simulink model "foc_im_spwm"  (R2024b)
settings: Solver=FixedStepDiscrete  StartTime=0.0  StopTime=P.T_end  FixedStep=P.Ts_power  RelTol=1e-3
values from neighbouring files (symbols this model uses):
  P = motor_params()    [compare_foc_pwm.m]
undefined symbols (not defined in the file or in its folder): DiscIntNeverNeededParam
libraries: slpidlib x3, spsCurrentMeasurementLib x2, spsGroundLib x1, spsabctodq0Lib x1, spsdq0toabcLib x1, spsAsynchronousMachineSIUnitsLib x1, spsUniversalBridgeLib x1, spsDCVoltageSourceLib x1, spspowerguiLib x1
settings Model: Creator=khali  LastModifiedBy=Khalil
settings SolverCC: AutoInsertRateTranBlk=on

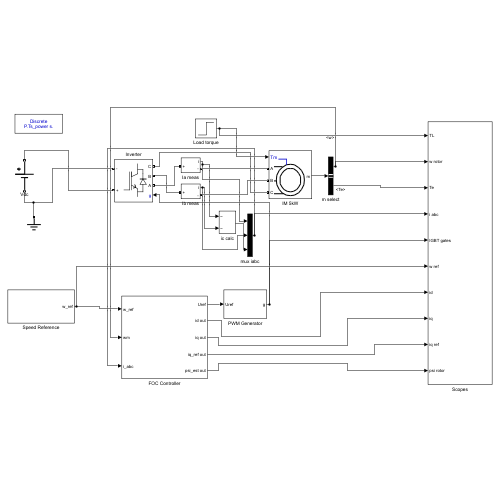
[thumbnail: Simulink's stored preview of the top-level diagram]
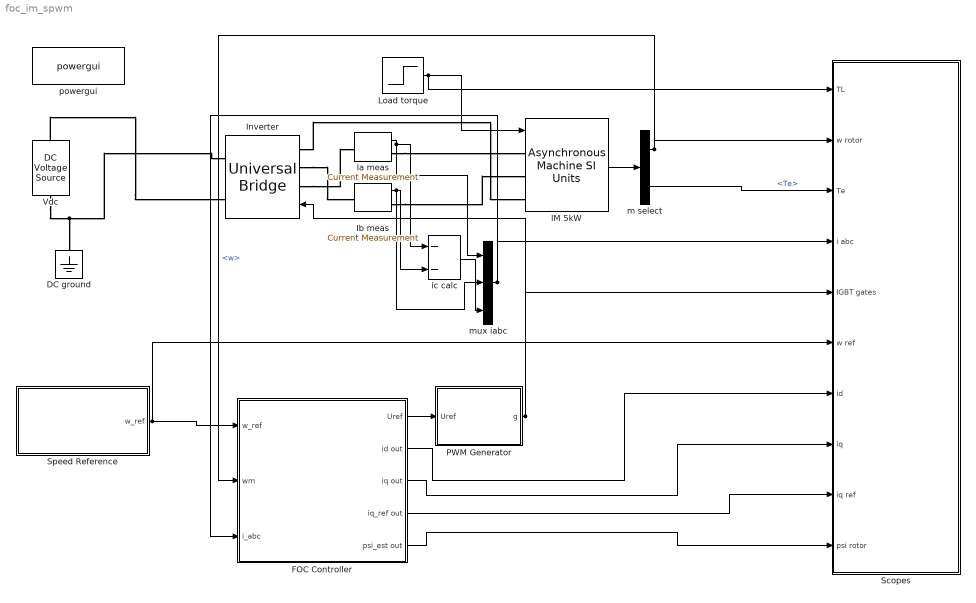
== system foc_im_spwm ==
  DC ground : spsGroundLib/Ground  LConnTagsString=a
  FOC Controller : Subsystem
  IM 5kW : spsAsynchronousMachineSIUnitsLib/Asynchronous Machine SI Units  RotorType=Squirrel-cage  PresetModel=No  MechanicalLoad=Torque Tm  ShowDetailedParameters=on  ReferenceFrame=Rotor  Units=SI  MeasurementBus=on  NominalParameters=[P.Pn P.Vn P.fn]  VoltageRatio=1  Stator=[P.Rs P.Lls]  Rotor=[P.Rr P.Llr]  Cage1=[0.4155 0.002066]  Cage2=[0.4168 0.0003495]  Lm=P.Lm  Mechanical=[P.J P.B P.p]  PolePairs=2  InitialConditions=[1 0 0 0 0 0 0 0]  SimulateSaturation=off  Saturation=[14.03593122, 27.81365428, 53.79336849, 72.68890987, 97.98006896, 148.6815601, 215.7428561, 302.9841135, 428.7778367 ; 230, 322, 414, 460, 506, 552, 598, 644, 690]  LoadFlowParameters=1492000  TsPowergui=0  TsBlock=-1  IterativeModel=Trapezoidal non iterative  IterativeDiscreteModel=Trapezoidal non iterative  Pmec=1.492e+006
  Ia meas : spsCurrentMeasurementLib/Current Measurement  PhasorSimulation=off  OutputType=Complex  PSBequivalent=0
  Ib meas : spsCurrentMeasurementLib/Current Measurement  PhasorSimulation=off  OutputType=Complex  PSBequivalent=0
  Inverter : spsUniversalBridgeLib/Universal Bridge  Arms=3  SnubberResistance=1e5  SnubberCapacitance=inf  Device=IGBT / Diodes  Ron=1e-3  Lon=0  ForwardVoltages="[  0  0  ]"  ForwardVoltage=0  GTOparameters=[ 10e-6 , 20e-6 ]  IGBTparameters=[ 1e-6 , 2e-6 ]  Measurements=None  Measurements_2=None  converterType=Inverter
  Load torque : Step  Time=P.t_load  After=P.TL  SampleTime=0
  PWM Generator : Subsystem
  Scopes : Subsystem
  Speed Reference : Subsystem
  Vdc : spsDCVoltageSourceLib/DC Voltage Source  Amplitude=P.Vdc  Measurements=None
  ic calc : Sum  Inputs=--
  m select : BusSelector  OutputSignals=w,Te
  mux iabc : Mux  Inputs=3
  powergui : spspowerguiLib/powergui  Priority=1  SimulationMode=Discrete  SampleTime=P.Ts_power  frequency=60  Iterations=50  frequencyindice=50  Pbase=100e6  ErrMax=1e-4  UnitsV=kV  UnitsW=MW  buscounter=0  FunctionMessages=off  echomessages=off  EnableUseOfTLC=off  CurrentSourceSwitches=off  DisableSnubberDevices=off  DisableRonSwitches=off  DisableVfSwitches=off  DisplayEquations=off  AutomaticDiscreteSolvers=off  SolverType=Tustin/Backward Euler (TBE)  Interpol=off  ExternalGateDelay=off  methode=off  Ts=100  x0status=blocks  SPID=on  SwTol=0  HookPort=off  NonlinearTolerance=1e-4  nMaxIteration=100  ContinueOnMaxIteration=off  RestoreLinks=warning  ResistiveCurrentMeasurement=off  Frange=[0:2:500]  Ylog=off  Xlog=on  ShowGrid=off  save=off  variable=ZData  structure=0  ZoomFFT=off  StartTime=0.0  cycles=1  DisplayStyle=1  fundamental=60  FreqAxis=off  MaxFrequency=1000  frequencyindicesteady=1  RmsSteady=1  display=off
  wires:
  Ia meas/1 -> ic calc/1, mux iabc/1
  Ib meas/1 -> ic calc/2, mux iabc/2
  ic calc/1 -> mux iabc/3
  Speed Reference/1(w_ref) -> FOC Controller/1(w_ref), Scopes/6(w ref)
  Load torque/1 -> IM 5kW/1, Scopes/1(TL)
  IM 5kW/1 -> m select/1
  mux iabc/1 -> FOC Controller/3(i_abc), Scopes/4(i abc)
  m select/1 -> FOC Controller/2(wm), Scopes/2(w rotor)  "<w>"
  FOC Controller/1(Uref) -> PWM Generator/1(Uref)
  PWM Generator/1(g) -> Inverter/1, Scopes/5(IGBT gates)
  m select/2 -> Scopes/3(Te)  "<Te>"
  FOC Controller/2(id out) -> Scopes/7(id)
  FOC Controller/3(iq out) -> Scopes/8(iq)
  FOC Controller/4(iq_ref out) -> Scopes/9(iq ref)
  FOC Controller/5(psi_est out) -> Scopes/10(psi rotor)
  connections:
  Vdc/RConn1 -- Inverter/RConn1
  Inverter/RConn2 -- Vdc/LConn1 -- DC ground/LConn1
  Inverter/LConn1 -- Ia meas/LConn1
  Inverter/LConn2 -- Ib meas/LConn1
  Ia meas/RConn1 -- IM 5kW/LConn1
  Ib meas/RConn1 -- IM 5kW/LConn2
  Inverter/LConn3 -- IM 5kW/LConn3

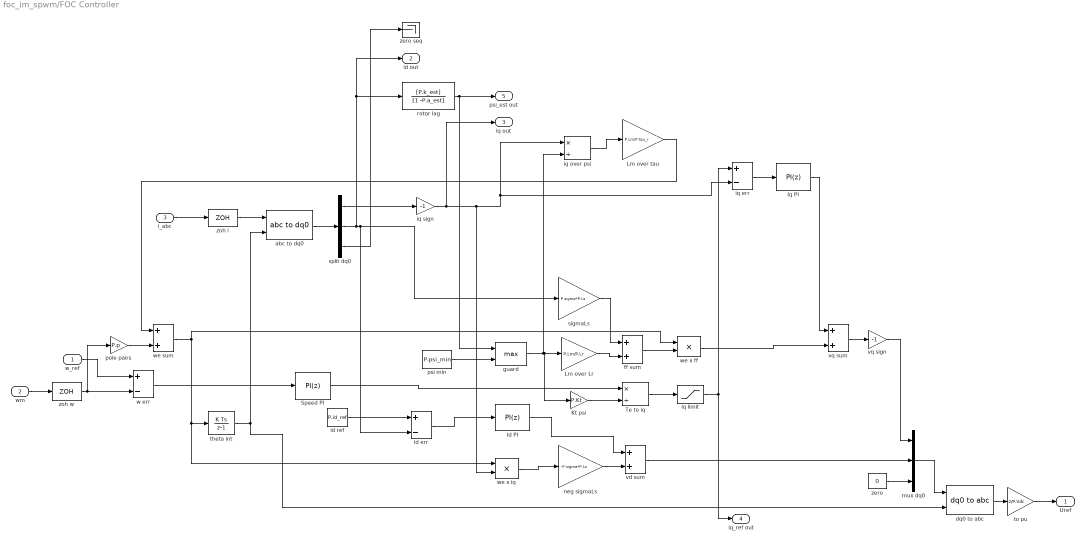
== system foc_im_spwm/FOC Controller ==
  w_ref : Inport
  wm : Inport  Port=2
  i_abc : Inport  Port=3
  Id PI : slpidlib/PID Controller  Controller=PI  Form=Parallel  TimeDomain=Discrete-time  UseExternalTs=off  SampleTime=P.Ts_ctrl  IntegratorMethod=Forward Euler  FilterMethod=Forward Euler  ControllerParametersSource=internal  P=P.Kp_i  I=P.Ki_i  UseKiTs=off  D=0  UseExternalDerivativeSource=off  N=100  UseFilter=on  TunerSelectOption=Transfer Function Based (PID Tuner App)  InitialConditionSource=internal  InitialConditionForIntegrator=0  InitialConditionForFilter=0  DifferentiatorICPrevScaledInput=0  ExternalReset=none  TrackingMode=off  Kt=1  LimitOutput=on  SatLimitsSource=internal  UpperSaturationLimit=P.v_max  LowerSaturationLimit=-P.v_max  LinearizeAsGain=on  AntiWindupMode=clamping  Kb=1  LimitIntegrator=off  UpperIntegratorSaturationLimit=inf  LowerIntegratorSaturationLimit=-inf  POutMin=[]  POutMax=[]  IOutMin=[]  IOutMax=[]  DOutMin=[]  DOutMax=[]  NOutMin=[]  NOutMax=[]  SumOutMin=[]  SumOutMax=[]  SaturationOutMin=[]  SaturationOutMax=[]  PParamMin=[]  PParamMax=[]  IParamMin=[]  IParamMax=[]  DParamMin=[]  DParamMax=[]  NParamMin=[]  NParamMax=[]  KbParamMin=[]  KbParamMax=[]  KtParamMin=[]  KtParamMax=[]  KbOutMin=[]  KbOutMax=[]  KtOutMin=[]  KtOutMax=[]  IntegratorOutMin=[]  IntegratorOutMax=[]  FilterOutMin=[]  FilterOutMax=[]  SumI1OutMin=[]  SumI1OutMax=[]  SumI2OutMin=[]  SumI2OutMax=[]  SumI3OutMin=[]  SumI3OutMax=[]  SumI4OutMin=[]  SumI4OutMax=[]  SumDOutMin=[]  SumDOutMax=[]  DifferentiatorOutMin=[]  DifferentiatorOutMax=[]  FilterDiffOutCoefMin=[]  FilterDiffOutCoefMax=[]  ReciprocalOutMin=[]  ReciprocalOutMax=[]  SumDenOutMin=[]  SumDenOutMax=[]  SumNumOutMin=[]  SumNumOutMax=[]  DivideOutMin=[]  DivideOutMax=[]  UdiffTsProdOutMin=[]  UdiffTsProdOutMax=[]  NTsProdOutMin=[]  NTsProdOutMax=[]  UintegralTsProdOutMin=[]  UintegralTsProdOutMax=[]  UngainTsProdOutMin=[]  UngainTsProdOutMax=[]  ClampingZeroOutDataTypeStr=Inherit: Inherit via back propagation  ClampingZeroOutMin=[]  ClampingZeroOutMax=[]  FilterDenConstantOutDataTypeStr=Inherit: Inherit via back propagation  FilterDenConstantOutMin=[]  FilterDenConstantOutMax=[]  PCopyOutDataTypeStr=Inherit: Inherit via back propagation  PCopyOutMin=[]  PCopyOutMax=[]  NCopyOutDataTypeStr=Inherit: Inherit via back propagation  NCopyOutMin=[]  NCopyOutMax=[]  IntegratorContinuousStateAttributes=''  IntegratorStateMustResolveToSignalObject=off  IntegratorRTWStateStorageClass=Auto  FilterContinuousStateAttributes=''  FilterStateMustResolveToSignalObject=off  FilterRTWStateStorageClass=Auto  ParallelPVariant=InternalParameters  IdealPVariant=Disabled  IVariant=InternalParameters  DVariant=Disabled  IntegratorVariant=Discrete  SatVariant=Enabled  AWVariant=DiscClampingParallel  PCopyVariant=Disabled  TRVariant=Disabled  FdbkBlocksVariant=Forward  IdealPFdbkVariant=Disabled  SatFdbkVariant=Disabled  DerivativeFilterVariant=Disabled  NVariant=Disabled  NCopyVariant=Disabled_SignalSpec  FilterICVariant=Disabled  IntegratorICVariant=InternalICs  ExternalResetVariant=Disabled  TRSumVariant=Passthrough  SumFdbkVariant=Disabled  SumVariant=Sum_PI  TsampFilterVariant=InternalTs  TsampNgainVariant=Passthrough  TsampIntegralVariant=Disabled_SignalSpec  ExternalSaturationOutDataTypeStr=Inherit: Same as second input  DerivativeSourceVariant=Disabled  PreIntVariant=InternalPreInt
  Iq PI : slpidlib/PID Controller  Controller=PI  Form=Parallel  TimeDomain=Discrete-time  UseExternalTs=off  SampleTime=P.Ts_ctrl  IntegratorMethod=Forward Euler  FilterMethod=Forward Euler  ControllerParametersSource=internal  P=P.Kp_i  I=P.Ki_i  UseKiTs=off  D=0  UseExternalDerivativeSource=off  N=100  UseFilter=on  TunerSelectOption=Transfer Function Based (PID Tuner App)  InitialConditionSource=internal  InitialConditionForIntegrator=0  InitialConditionForFilter=0  DifferentiatorICPrevScaledInput=0  ExternalReset=none  TrackingMode=off  Kt=1  LimitOutput=on  SatLimitsSource=internal  UpperSaturationLimit=P.v_max  LowerSaturationLimit=-P.v_max  LinearizeAsGain=on  AntiWindupMode=clamping  Kb=1  LimitIntegrator=off  UpperIntegratorSaturationLimit=inf  LowerIntegratorSaturationLimit=-inf  POutMin=[]  POutMax=[]  IOutMin=[]  IOutMax=[]  DOutMin=[]  DOutMax=[]  NOutMin=[]  NOutMax=[]  SumOutMin=[]  SumOutMax=[]  SaturationOutMin=[]  SaturationOutMax=[]  PParamMin=[]  PParamMax=[]  IParamMin=[]  IParamMax=[]  DParamMin=[]  DParamMax=[]  NParamMin=[]  NParamMax=[]  KbParamMin=[]  KbParamMax=[]  KtParamMin=[]  KtParamMax=[]  KbOutMin=[]  KbOutMax=[]  KtOutMin=[]  KtOutMax=[]  IntegratorOutMin=[]  IntegratorOutMax=[]  FilterOutMin=[]  FilterOutMax=[]  SumI1OutMin=[]  SumI1OutMax=[]  SumI2OutMin=[]  SumI2OutMax=[]  SumI3OutMin=[]  SumI3OutMax=[]  SumI4OutMin=[]  SumI4OutMax=[]  SumDOutMin=[]  SumDOutMax=[]  DifferentiatorOutMin=[]  DifferentiatorOutMax=[]  FilterDiffOutCoefMin=[]  FilterDiffOutCoefMax=[]  ReciprocalOutMin=[]  ReciprocalOutMax=[]  SumDenOutMin=[]  SumDenOutMax=[]  SumNumOutMin=[]  SumNumOutMax=[]  DivideOutMin=[]  DivideOutMax=[]  UdiffTsProdOutMin=[]  UdiffTsProdOutMax=[]  NTsProdOutMin=[]  NTsProdOutMax=[]  UintegralTsProdOutMin=[]  UintegralTsProdOutMax=[]  UngainTsProdOutMin=[]  UngainTsProdOutMax=[]  ClampingZeroOutDataTypeStr=Inherit: Inherit via back propagation  ClampingZeroOutMin=[]  ClampingZeroOutMax=[]  FilterDenConstantOutDataTypeStr=Inherit: Inherit via back propagation  FilterDenConstantOutMin=[]  FilterDenConstantOutMax=[]  PCopyOutDataTypeStr=Inherit: Inherit via back propagation  PCopyOutMin=[]  PCopyOutMax=[]  NCopyOutDataTypeStr=Inherit: Inherit via back propagation  NCopyOutMin=[]  NCopyOutMax=[]  IntegratorContinuousStateAttributes=''  IntegratorStateMustResolveToSignalObject=off  IntegratorRTWStateStorageClass=Auto  FilterContinuousStateAttributes=''  FilterStateMustResolveToSignalObject=off  FilterRTWStateStorageClass=Auto  ParallelPVariant=InternalParameters  IdealPVariant=Disabled  IVariant=InternalParameters  DVariant=Disabled  IntegratorVariant=Discrete  SatVariant=Enabled  AWVariant=DiscClampingParallel  PCopyVariant=Disabled  TRVariant=Disabled  FdbkBlocksVariant=Forward  IdealPFdbkVariant=Disabled  SatFdbkVariant=Disabled  DerivativeFilterVariant=Disabled  NVariant=Disabled  NCopyVariant=Disabled_SignalSpec  FilterICVariant=Disabled  IntegratorICVariant=InternalICs  ExternalResetVariant=Disabled  TRSumVariant=Passthrough  SumFdbkVariant=Disabled  SumVariant=Sum_PI  TsampFilterVariant=InternalTs  TsampNgainVariant=Passthrough  TsampIntegralVariant=Disabled_SignalSpec  ExternalSaturationOutDataTypeStr=Inherit: Same as second input  DerivativeSourceVariant=Disabled  PreIntVariant=InternalPreInt
  Kt psi : Gain  Gain=P.Kt
  Lm over Lr : Gain  Gain=P.Lm/P.Lr
  Lm over tau : Gain  Gain=P.Lm/P.tau_r
  Speed PI : slpidlib/PID Controller  Controller=PI  Form=Parallel  TimeDomain=Discrete-time  UseExternalTs=off  SampleTime=P.Ts_ctrl  IntegratorMethod=Forward Euler  FilterMethod=Forward Euler  ControllerParametersSource=internal  P=P.Kp_w  I=P.Ki_w  UseKiTs=off  D=0  UseExternalDerivativeSource=off  N=100  UseFilter=on  TunerSelectOption=Transfer Function Based (PID Tuner App)  InitialConditionSource=internal  InitialConditionForIntegrator=0  InitialConditionForFilter=0  DifferentiatorICPrevScaledInput=0  ExternalReset=none  TrackingMode=off  Kt=1  LimitOutput=on  SatLimitsSource=internal  UpperSaturationLimit=P.Te_max  LowerSaturationLimit=-P.Te_max  LinearizeAsGain=on  AntiWindupMode=clamping  Kb=1  LimitIntegrator=off  UpperIntegratorSaturationLimit=inf  LowerIntegratorSaturationLimit=-inf  POutMin=[]  POutMax=[]  IOutMin=[]  IOutMax=[]  DOutMin=[]  DOutMax=[]  NOutMin=[]  NOutMax=[]  SumOutMin=[]  SumOutMax=[]  SaturationOutMin=[]  SaturationOutMax=[]  PParamMin=[]  PParamMax=[]  IParamMin=[]  IParamMax=[]  DParamMin=[]  DParamMax=[]  NParamMin=[]  NParamMax=[]  KbParamMin=[]  KbParamMax=[]  KtParamMin=[]  KtParamMax=[]  KbOutMin=[]  KbOutMax=[]  KtOutMin=[]  KtOutMax=[]  IntegratorOutMin=[]  IntegratorOutMax=[]  FilterOutMin=[]  FilterOutMax=[]  SumI1OutMin=[]  SumI1OutMax=[]  SumI2OutMin=[]  SumI2OutMax=[]  SumI3OutMin=[]  SumI3OutMax=[]  SumI4OutMin=[]  SumI4OutMax=[]  SumDOutMin=[]  SumDOutMax=[]  DifferentiatorOutMin=[]  DifferentiatorOutMax=[]  FilterDiffOutCoefMin=[]  FilterDiffOutCoefMax=[]  ReciprocalOutMin=[]  ReciprocalOutMax=[]  SumDenOutMin=[]  SumDenOutMax=[]  SumNumOutMin=[]  SumNumOutMax=[]  DivideOutMin=[]  DivideOutMax=[]  UdiffTsProdOutMin=[]  UdiffTsProdOutMax=[]  NTsProdOutMin=[]  NTsProdOutMax=[]  UintegralTsProdOutMin=[]  UintegralTsProdOutMax=[]  UngainTsProdOutMin=[]  UngainTsProdOutMax=[]  ClampingZeroOutDataTypeStr=Inherit: Inherit via back propagation  ClampingZeroOutMin=[]  ClampingZeroOutMax=[]  FilterDenConstantOutDataTypeStr=Inherit: Inherit via back propagation  FilterDenConstantOutMin=[]  FilterDenConstantOutMax=[]  PCopyOutDataTypeStr=Inherit: Inherit via back propagation  PCopyOutMin=[]  PCopyOutMax=[]  NCopyOutDataTypeStr=Inherit: Inherit via back propagation  NCopyOutMin=[]  NCopyOutMax=[]  IntegratorContinuousStateAttributes=''  IntegratorStateMustResolveToSignalObject=off  IntegratorRTWStateStorageClass=Auto  FilterContinuousStateAttributes=''  FilterStateMustResolveToSignalObject=off  FilterRTWStateStorageClass=Auto  ParallelPVariant=InternalParameters  IdealPVariant=Disabled  IVariant=InternalParameters  DVariant=Disabled  IntegratorVariant=Discrete  SatVariant=Enabled  AWVariant=DiscClampingParallel  PCopyVariant=Disabled  TRVariant=Disabled  FdbkBlocksVariant=Forward  IdealPFdbkVariant=Disabled  SatFdbkVariant=Disabled  DerivativeFilterVariant=Disabled  NVariant=Disabled  NCopyVariant=Disabled_SignalSpec  FilterICVariant=Disabled  IntegratorICVariant=InternalICs  ExternalResetVariant=Disabled  TRSumVariant=Passthrough  SumFdbkVariant=Disabled  SumVariant=Sum_PI  TsampFilterVariant=InternalTs  TsampNgainVariant=Passthrough  TsampIntegralVariant=Disabled_SignalSpec  ExternalSaturationOutDataTypeStr=Inherit: Same as second input  DerivativeSourceVariant=Disabled  PreIntVariant=InternalPreInt
  Te to iq : Product  Inputs=*/
  abc to dq0 : spsabctodq0Lib/abc to dq0  Alignment=90 degrees behind phase A axis
  dq0 to abc : spsdq0toabcLib/dq0 to abc  Alignment=90 degrees behind phase A axis
  ff sum : Sum
  guard : MinMax  Function=max  Inputs=2
  id err : Sum  Inputs=+-
  id ref : Constant  Value=P.id_ref
  iq err : Sum  Inputs=+-
  iq limit : Saturate  UpperLimit=P.iq_max  LowerLimit=-P.iq_max
  iq over psi : Product  Inputs=*/
  iq sign : Gain  Gain=-1
  mux dq0 : Mux  Inputs=3
  neg sigmaLs : Gain  Gain=-P.sigma*P.Ls
  pole pairs : Gain  Gain=P.p
  psi min : Constant  Value=P.psi_min
  rotor lag : DiscreteTransferFcn  Numerator=[P.k_est]  Denominator=[1 -P.a_est]  SampleTime=P.Ts_ctrl
  sigmaLs : Gain  Gain=P.sigma*P.Ls
  split dq0 : Demux  Outputs=3
  theta int : DiscreteIntegrator  SampleTime=P.Ts_ctrl  ICPrevOutput=DiscIntNeverNeededParam  ICPrevScaledInput=DiscIntNeverNeededParam
  to pu : Gain  Gain=2/P.Vdc
  vd sum : Sum
  vq sign : Gain  Gain=-1
  vq sum : Sum
  w err : Sum  Inputs=+-
  we sum : Sum
  we x ff : Product
  we x iq : Product
  zero : Constant  Value=0
  zero seq : Terminator
  zoh i : ZeroOrderHold  SampleTime=P.Ts_ctrl
  zoh w : ZeroOrderHold  SampleTime=P.Ts_ctrl
  Uref : Outport
  id out : Outport  Port=2
  iq out : Outport  Port=3
  iq_ref out : Outport  Port=4
  psi_est out : Outport  Port=5
  wires:
  Kt psi/1 -> Te to iq/2
  zoh i/1 -> abc to dq0/1
  i_abc/1 -> zoh i/1
  w err/1 -> Speed PI/1
  w_ref/1 -> w err/1
  Te to iq/1 -> iq limit/1
  wm/1 -> zoh w/1
  iq sign/1 -> iq over psi/1, iq err/2, we x iq/2, iq out/1
  zoh w/1 -> pole pairs/1, w err/2
  pole pairs/1 -> we sum/2
  we sum/1 -> we x iq/1, theta int/1, we x ff/1
  theta int/1 -> dq0 to abc/2, abc to dq0/2
  abc to dq0/1 -> split dq0/1
  split dq0/3 -> zero seq/1
  Speed PI/1 -> Te to iq/1
  sigmaLs/1 -> ff sum/1
  split dq0/1 -> iq sign/1
  dq0 to abc/1 -> to pu/1
  vq sign/1 -> mux dq0/1
  split dq0/2 -> sigmaLs/1, id err/2, rotor lag/1, id out/1
  id err/1 -> Id PI/1
  id ref/1 -> id err/1
  rotor lag/1 -> guard/1, psi_est out/1
  psi min/1 -> guard/2
  guard/1 -> Kt psi/1, Lm over Lr/1, iq over psi/2
  Id PI/1 -> vd sum/1
  we x iq/1 -> neg sigmaLs/1
  iq over psi/1 -> Lm over tau/1
  we x ff/1 -> vq sum/2
  vd sum/1 -> mux dq0/2
  Lm over Lr/1 -> ff sum/2
  neg sigmaLs/1 -> vd sum/2
  Lm over tau/1 -> we sum/1
  vq sum/1 -> vq sign/1
  ff sum/1 -> we x ff/2
  iq limit/1 -> iq err/1, iq_ref out/1
  iq err/1 -> Iq PI/1
  Iq PI/1 -> vq sum/1
  to pu/1 -> Uref/1
  zero/1 -> mux dq0/3
  mux dq0/1 -> dq0 to abc/1

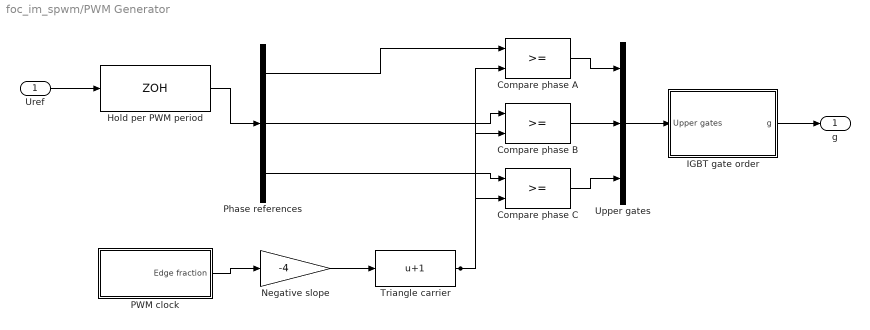
== system foc_im_spwm/PWM Generator ==
  Uref : Inport  PortDimensions=3
  Compare phase A : RelationalOperator  OutDataTypeStr=boolean  RndMeth=Simplest  InputSameDT=off
  Compare phase B : RelationalOperator  OutDataTypeStr=boolean  RndMeth=Simplest  InputSameDT=off
  Compare phase C : RelationalOperator  OutDataTypeStr=boolean  RndMeth=Simplest  InputSameDT=off
  Hold per PWM period : ZeroOrderHold  SampleTime=1/P.fsw
  IGBT gate order : Subsystem
  Negative slope : Gain  Gain=-4
  PWM clock : Subsystem
  Phase references : Demux  Outputs=3
  Triangle carrier : Bias  Bias=1  SaturateOnIntegerOverflow=off
  Upper gates : Mux  Inputs=3
  g : Outport
  wires:
  Phase references/1 -> Compare phase A/1
  Triangle carrier/1 -> Compare phase A/2, Compare phase B/2, Compare phase C/2
  Phase references/2 -> Compare phase B/1
  Phase references/3 -> Compare phase C/1
  Uref/1 -> Hold per PWM period/1
  Hold per PWM period/1 -> Phase references/1
  PWM clock/1(Edge fraction) -> Negative slope/1
  Negative slope/1 -> Triangle carrier/1
  Compare phase A/1 -> Upper gates/1
  Compare phase B/1 -> Upper gates/2
  Compare phase C/1 -> Upper gates/3
  Upper gates/1 -> IGBT gate order/1(Upper gates)
  IGBT gate order/1(g) -> g/1

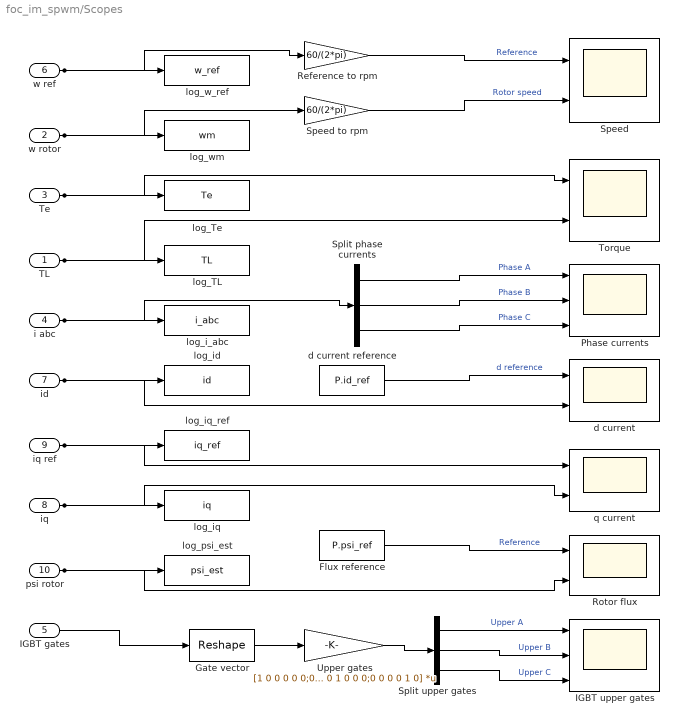
== system foc_im_spwm/Scopes ==
  TL : Inport
  w rotor : Inport  Port=2
  Te : Inport  Port=3
  i abc : Inport  Port=4
  IGBT gates : Inport  Port=5
  w ref : Inport  Port=6
  id : Inport  Port=7
  iq : Inport  Port=8
  iq ref : Inport  Port=9
  psi rotor : Inport  Port=10
  Flux reference : Constant  Value=P.psi_ref
  Gate vector : Reshape
  IGBT upper gates : Scope  NumInputPorts=3
  Phase currents : Scope  NumInputPorts=3
  Reference to rpm : Gain  Gain=60/(2*pi)
  Rotor flux : Scope  NumInputPorts=2
  Speed : Scope  NumInputPorts=2
  Speed to rpm : Gain  Gain=60/(2*pi)
  Split phase currents : Demux  Outputs=3
  Split upper gates : Demux  Outputs=3
  Torque : Scope  NumInputPorts=2
  Upper gates : Gain  Gain=[1 0 0 0 0 0;0 0 1 0 0 0;0 0 0 0 1 0]  Multiplication=Matrix(K*u)
  d current : Scope  NumInputPorts=2
  d current reference : Constant  Value=P.id_ref
  log_TL : ToWorkspace  VariableName=TL  SaveFormat=Timeseries  SampleTime=-1
  log_Te : ToWorkspace  VariableName=Te  SaveFormat=Timeseries  SampleTime=-1
  log_i_abc : ToWorkspace  VariableName=i_abc  SaveFormat=Timeseries  SampleTime=-1
  log_id : ToWorkspace  VariableName=id  SaveFormat=Timeseries  SampleTime=-1
  log_iq : ToWorkspace  VariableName=iq  SaveFormat=Timeseries  SampleTime=-1
  log_iq_ref : ToWorkspace  VariableName=iq_ref  SaveFormat=Timeseries  SampleTime=-1
  log_psi_est : ToWorkspace  VariableName=psi_est  SaveFormat=Timeseries  SampleTime=-1
  log_w_ref : ToWorkspace  VariableName=w_ref  SaveFormat=Timeseries  SampleTime=-1
  log_wm : ToWorkspace  VariableName=wm  SaveFormat=Timeseries  SampleTime=-1
  q current : Scope  NumInputPorts=2
  wires:
  TL/1 -> log_TL/1, Torque/2
  w rotor/1 -> log_wm/1, Speed to rpm/1
  Te/1 -> log_Te/1, Torque/1
  i abc/1 -> log_i_abc/1, Split phase currents/1
  w ref/1 -> log_w_ref/1, Reference to rpm/1
  id/1 -> log_id/1, d current/2
  iq/1 -> log_iq/1, q current/2
  iq ref/1 -> log_iq_ref/1, q current/1
  psi rotor/1 -> log_psi_est/1, Rotor flux/2
  Reference to rpm/1 -> Speed/1  "Reference"
  Speed to rpm/1 -> Speed/2  "Rotor speed"
  Split phase currents/1 -> Phase currents/1  "Phase A"
  Split phase currents/2 -> Phase currents/2  "Phase B"
  Split phase currents/3 -> Phase currents/3  "Phase C"
  d current reference/1 -> d current/1  "d reference"
  Flux reference/1 -> Rotor flux/1  "Reference"
  IGBT gates/1 -> Gate vector/1
  Gate vector/1 -> Upper gates/1
  Upper gates/1 -> Split upper gates/1
  Split upper gates/1 -> IGBT upper gates/1  "Upper A"
  Split upper gates/2 -> IGBT upper gates/2  "Upper B"
  Split upper gates/3 -> IGBT upper gates/3  "Upper C"

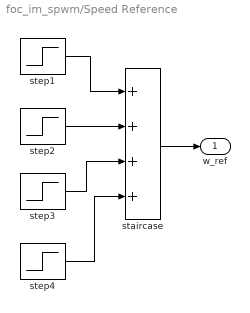
== system foc_im_spwm/Speed Reference ==
  staircase : Sum  Inputs=++++
  step1 : Step  Time=P.step_t(1)  After=P.step_d(1)  SampleTime=0
  step2 : Step  Time=P.step_t(2)  After=P.step_d(2)  SampleTime=0
  step3 : Step  Time=P.step_t(3)  After=P.step_d(3)  SampleTime=0
  step4 : Step  Time=P.step_t(4)  After=P.step_d(4)  SampleTime=0
  w_ref : Outport
  wires:
  staircase/1 -> w_ref/1
  step4/1 -> staircase/4
  step3/1 -> staircase/3
  step2/1 -> staircase/2
  step1/1 -> staircase/1

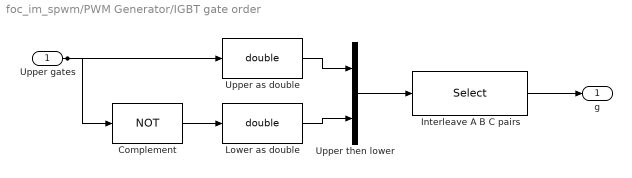
== system foc_im_spwm/PWM Generator/IGBT gate order ==
  Upper gates : Inport
  Complement : Logic  Operator=NOT  AllPortsSameDT=off  OutDataTypeStr=boolean
  Interleave A B C pairs : Selector  InputPortWidth=6  IndexOptions=Index vector (dialog)  Indices=[1 4 2 5 3 6]  OutputSizes=1
  Lower as double : DataTypeConversion  OutDataTypeStr=double  SaturateOnIntegerOverflow=off  RndMeth=Floor
  Upper as double : DataTypeConversion  OutDataTypeStr=double  SaturateOnIntegerOverflow=off  RndMeth=Floor
  Upper then lower : Mux  Inputs=2
  g : Outport
  wires:
  Upper gates/1 -> Complement/1, Upper as double/1
  Complement/1 -> Lower as double/1
  Upper as double/1 -> Upper then lower/1
  Lower as double/1 -> Upper then lower/2
  Upper then lower/1 -> Interleave A B C pairs/1
  Interleave A B C pairs/1 -> g/1

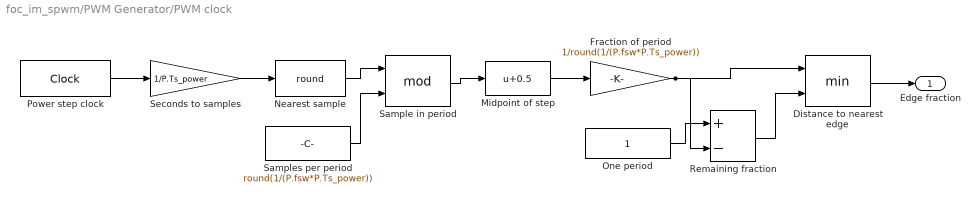
== system foc_im_spwm/PWM Generator/PWM clock ==
  Distance to nearest edge : MinMax  Inputs=2
  Fraction of period : Gain  Gain=1/round(1/(P.fsw*P.Ts_power))
  Midpoint of step : Bias  Bias=0.5  SaturateOnIntegerOverflow=off
  Nearest sample : Rounding  Operator=round
  One period : Constant
  Power step clock : DigitalClock  SampleTime=P.Ts_power
  Remaining fraction : Sum  Inputs=+-
  Sample in period : Math  Operator=mod
  Samples per period : Constant  Value=round(1/(P.fsw*P.Ts_power))
  Seconds to samples : Gain  Gain=1/P.Ts_power
  Edge fraction : Outport
  wires:
  Power step clock/1 -> Seconds to samples/1
  Seconds to samples/1 -> Nearest sample/1
  Nearest sample/1 -> Sample in period/1
  Samples per period/1 -> Sample in period/2
  Sample in period/1 -> Midpoint of step/1
  Midpoint of step/1 -> Fraction of period/1
  One period/1 -> Remaining fraction/1
  Fraction of period/1 -> Remaining fraction/2, Distance to nearest edge/1
  Remaining fraction/1 -> Distance to nearest edge/2
  Distance to nearest edge/1 -> Edge fraction/1
